simulink model "FSI_2DOF_Simscape"  (R2024a)
settings: Solver=FixedStepAuto  StartTime=0.0  StopTime=30  FixedStep=1e-4  MaxStep=1e-5  MinStep=1e-5  RelTol=1e-6  EnableMultiTasking=on
InitFcn:
  | FSI_2DOF_Simscape_init
values from neighbouring files (symbols this model uses):
  b1 = 1.5e2    (= 150)    [FSI_2DOF_Simscape_init.m]
  b2 = 5    [FSI_2DOF_Simscape_init.m]
  bias_1 = 0    [FSI_2DOF_Simscape_init.m]
  bias_2 = 0    [FSI_2DOF_Simscape_init.m]
  F_1 = 1e4    (= 10000)    [FSI_2DOF_Simscape_init.m]
  F_2 = 0    [FSI_2DOF_Simscape_init.m]
  omega_1 = 2*pi*f_1    [FSI_2DOF_Simscape_init.m]
  omega_2 = 2*pi*f_2    [FSI_2DOF_Simscape_init.m]
  phase_1 = 0    [FSI_2DOF_Simscape_init.m]
  phase_2 = 0    [FSI_2DOF_Simscape_init.m]
  t_1 = 1e-2    (= 0.01)    [FSI_2DOF_Simscape_init.m]
  t_2 = 1e-2    (= 0.01)    [FSI_2DOF_Simscape_init.m]
libraries: fl_lib x15, nesl_utility x7
settings Model: Creator=FilipKsica  LastModifiedBy=144901
settings SolverCC: InitialStep=1e-5  AlgebraicLoopSolver=TrustRegion
settings DataIOCC: LimitDataPoints=on  ReturnWorkspaceOutputs=off
settings OptimizationCC: LifeSpan=inf
settings DebuggingCC: UnconnectedInputMsg=warning  UnconnectedOutputMsg=warning  UnconnectedLineMsg=warning  AllowSymbolicDim=off  SFUnexpectedBacktrackingDiag=warning  SFNoUnconditionalDefaultTransitionDiag=warning  SFExecutionAtInitializationDiag=none  ArithmeticOperatorsInVariantConditions=warning
settings ModelReferenceCC: EnableRefExpFcnMdlSchedulingChecks=on  PropagateSignalLabelsOutOfModel=off
settings SFSimCC: SimUseLocalCustomCode=off  CustomCodeUndefinedFunction=UseInterfaceOnly
settings RTWCC: RTWUseLocalCustomCode=off  GPUComputeCapability=3.5  DLArmComputeVersion=19.05
settings CodeAppCC: StateflowObjectComments=on
settings GRTTargetCC: TargetLangStandard=C89/C90 (ANSI)
settings ConfigComp: CovMetricSettings=dw  CovSaveCumulativeToWorkspaceVar=on  CovSaveSingleToWorkspaceVar=on  CovExternalEMLEnable=off
settings SimscapeCC: SimscapeNormalizeSystem=off

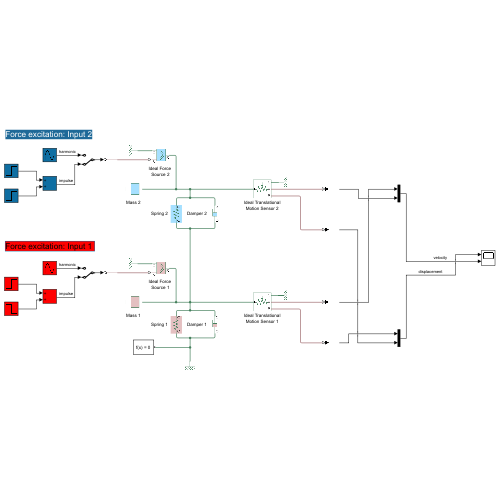
[thumbnail: Simulink's stored preview of the top-level diagram]
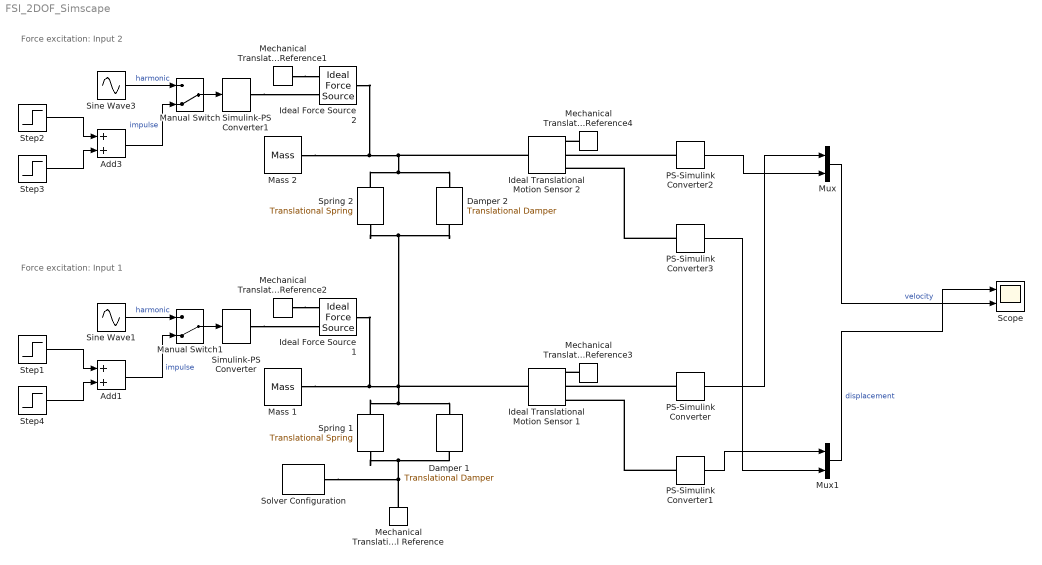
== system FSI_2DOF_Simscape ==
  note: Force excitation: Input 1
  note: Force excitation: Input 2
  Add1 : Sum
  Add3 : Sum
  Damper 1 : fl_lib/Mechanical/Translational Elements/Translational Damper  D=b1 N/(m/s)  v_specify=off  v_priority=None  v=0 m/s  v_nominal_specify=off  v_nominal_value=1  v_nominal_unit=m/s  f_specify=off  f_priority=None  f=0 N  f_nominal_specify=off  f_nominal_value=1  f_nominal_unit=N
  Damper 2 : fl_lib/Mechanical/Translational Elements/Translational Damper  D=b2 N/(m/s)  v_specify=off  v_priority=None  v=0 m/s  v_nominal_specify=off  v_nominal_value=1  v_nominal_unit=m/s  f_specify=off  f_priority=None  f=0 N  f_nominal_specify=off  f_nominal_value=1  f_nominal_unit=N
  Ideal Force Source 1 : fl_lib/Mechanical/Mechanical Sources/Ideal Force Source
  Ideal Force Source 2 : fl_lib/Mechanical/Mechanical Sources/Ideal Force Source
  Ideal Translational Motion Sensor 1 : fl_lib/Mechanical/Mechanical Sensors/Ideal Translational Motion Sensor  reference=foundation.enum.MeasurementReference.difference  acceleration_port=false  velocity_port=true  position_port=true  offset=0 m
  Ideal Translational Motion Sensor 2 : fl_lib/Mechanical/Mechanical Sensors/Ideal Translational Motion Sensor  reference=foundation.enum.MeasurementReference.difference  acceleration_port=false  velocity_port=true  position_port=true  offset=0 m
  Manual Switch : ManualSwitch  CurrentSetting=0
  Manual Switch1 : ManualSwitch  CurrentSetting=0
  Mass 1 : fl_lib/Mechanical/Translational Elements/Mass  mass=m1 kg  num_ports=foundation.enum.numPorts2.one  v_specify=off  v_priority=None  v=0 m/s  v_nominal_specify=off  v_nominal_value=1  v_nominal_unit=m/s  f_specify=off  f_priority=None  f=0 N  f_nominal_specify=off  f_nominal_value=1  f_nominal_unit=N
  Mass 2 : fl_lib/Mechanical/Translational Elements/Mass  mass=m2 kg  num_ports=foundation.enum.numPorts2.one  v_specify=off  v_priority=None  v=0 m/s  v_nominal_specify=off  v_nominal_value=1  v_nominal_unit=m/s  f_specify=off  f_priority=None  f=0 N  f_nominal_specify=off  f_nominal_value=1  f_nominal_unit=N
  Mechanical Translational Reference{,1..4} (5 alike) : fl_lib/Mechanical/Translational Elements/Mechanical Translational Reference
  Mux : Mux  Inputs=2
  Mux1 : Mux  Inputs=2
  PS-Simulink Converter{,1..3} (4 alike) : nesl_utility/PS-Simulink Converter  PhysicalDomain=network_engine_domain  SubClassName=ps_output  LeftPortType=input  RightPortType=output  PseudoPeriodic=off  Frequencies=[]  VectorFormat=1-D array  Unit=1  AffineConversion=off
  "Scope " : Scope  NumInputPorts=2
  Simulink-PS Converter : nesl_utility/Simulink-PS Converter  PhysicalDomain=network_engine_domain  SubClassName=ps_input  LeftPortType=input  RightPortType=output  PseudoPeriodic=off  Frequencies=[]  NoiseDistribution=none  NoiseParameters=[]  Unit=1  AffineConversion=off  FilteringAndDerivatives=zero  SimscapeFilterOrder=1  InputFilterTimeConstant=0.001  UdotUserProvided=1
  Simulink-PS Converter1 : nesl_utility/Simulink-PS Converter  PhysicalDomain=network_engine_domain  SubClassName=ps_input  LeftPortType=input  RightPortType=output  PseudoPeriodic=off  Frequencies=[]  NoiseDistribution=none  NoiseParameters=[]  Unit=1  AffineConversion=off  FilteringAndDerivatives=zero  SimscapeFilterOrder=1  InputFilterTimeConstant=0.001  UdotUserProvided=1
  Sine Wave1 : Sin  Amplitude=F_1  Bias=bias_1  Frequency=omega_1  Phase=phase_1  SampleTime=0
  Sine Wave3 : Sin  Amplitude=F_2  Bias=bias_2  Frequency=omega_2  Phase=phase_2  SampleTime=0
  Solver Configuration : nesl_utility/Solver Configuration  PhysicalDomain=network_engine_domain  SubClassName=solver  LeftPortType=input  RightPortType=generic  Tones=[]  Harmonics=[]  SimulateNoise=off  Profile=off  UseLocalSampling=off  EnableSwitchedLinearOptims=on  FrequencyDomain=off  UseCCode=off  RelTol=0.001  AbsTol=1e-06  MinStep=1e-09  ToWorkspace=off  RevertToSquareIcSolve=off  NumHomotopyIterations=100  PhasorMode=off  PhasorModeNumHarmonics=1  ConsistencySolver=NEWTON_FTOL  IndexReductionMethod=DerivativeReplacement  DoDC=off  ResidualTolerance=1e-09  ConsistencyTolSource=GLOBAL  ConsistencyAbsTol=0.001  ConsistencyRelTol=0.001  ConsistencyTolFactor=0.001  UseLocalSolver=off  LocalSolverChoice=NE_BACKWARD_EULER_ADVANCER  ResolveIndetEquations=on  FunctionEvalNumThread=1  LocalSolverSampleTime=0.001  DoFixedCost=off  MaxNonlinIter=3  MaxModeIter=2  ComputeImpulses=off  ImpulseIterations=2  LinearAlgebra=Sparse  LinearAlgebraNumThread=0  EquationFormulation=NE_TIME_EF  DelaysMemoryBudget=1024  AutomaticFiltering=on  FilteringTimeConstant=0.001  PartitionStorageMethod=AS_NEEDED  PartitionMemoryBudget=1024  PartitionMethod=FAST  MultibodyUseLocalSolver=off  MultibodyLocalSolverChoice=ODE1  MultibodyLocalSolverSampleTime=0.001
  Spring 1 : fl_lib/Mechanical/Translational Elements/Translational Spring  spr_rate=k1 N/m  v_specify=off  v_priority=None  v=0 m/s  v_nominal_specify=off  v_nominal_value=1  v_nominal_unit=m/s  f_specify=off  f_priority=None  f=0 N  f_nominal_specify=off  f_nominal_value=1  f_nominal_unit=N  x_specify=off  x_priority=None  x=0 m  x_nominal_specify=off  x_nominal_value=1  x_nominal_unit=m
  Spring 2 : fl_lib/Mechanical/Translational Elements/Translational Spring  spr_rate=k2 N/m  v_specify=off  v_priority=None  v=0 m/s  v_nominal_specify=off  v_nominal_value=1  v_nominal_unit=m/s  f_specify=off  f_priority=None  f=0 N  f_nominal_specify=off  f_nominal_value=1  f_nominal_unit=N  x_specify=off  x_priority=None  x=0 m  x_nominal_specify=off  x_nominal_value=1  x_nominal_unit=m
  Step1 : Step  Time=0  After=F_1  SampleTime=0
  Step2 : Step  Time=0  After=F_2  SampleTime=0
  Step3 : Step  Time=t_2  After=-F_2  SampleTime=0
  Step4 : Step  Time=t_1  After=-F_1  SampleTime=0
  wires:
  PS-Simulink Converter/1 -> Mux/1
  PS-Simulink Converter1/1 -> Mux1/1
  PS-Simulink Converter2/1 -> Mux/2
  PS-Simulink Converter3/1 -> Mux1/2
  Manual Switch1/1 -> Simulink-PS Converter/1
  Manual Switch/1 -> Simulink-PS Converter1/1
  Mux/1 -> "Scope "/2  "velocity"
  Mux1/1 -> "Scope "/1  "displacement"
  Step3/1 -> Add3/2
  Sine Wave3/1 -> Manual Switch/1  "harmonic"
  Add3/1 -> Manual Switch/2  "impulse"
  Step2/1 -> Add3/1
  Add1/1 -> Manual Switch1/2  "impulse"
  Step1/1 -> Add1/1
  Step4/1 -> Add1/2
  Sine Wave1/1 -> Manual Switch1/1  "harmonic"
  connections:
  Damper 2/RConn1 -- Spring 2/RConn1 -- Mass 1/LConn1 -- Ideal Force Source 1/LConn1 -- Ideal Translational Motion Sensor 1/LConn1 -- Spring 1/LConn1 -- Damper 1/LConn1
  Spring 1/RConn1 -- Solver Configuration/RConn1 -- Mechanical Translational Reference/LConn1 -- Damper 1/RConn1
  PS-Simulink Converter1/LConn1 -- Ideal Translational Motion Sensor 1/RConn3
  PS-Simulink Converter/LConn1 -- Ideal Translational Motion Sensor 1/RConn2
  Damper 2/LConn1 -- Ideal Translational Motion Sensor 2/LConn1 -- Mass 2/LConn1 -- Ideal Force Source 2/LConn1 -- Spring 2/LConn1
  Mechanical Translational Reference1/LConn1 -- Ideal Force Source 2/RConn2
  Mechanical Translational Reference2/LConn1 -- Ideal Force Source 1/RConn2
  Mechanical Translational Reference3/LConn1 -- Ideal Translational Motion Sensor 1/RConn1
  PS-Simulink Converter3/LConn1 -- Ideal Translational Motion Sensor 2/RConn3
  PS-Simulink Converter2/LConn1 -- Ideal Translational Motion Sensor 2/RConn2
  Mechanical Translational Reference4/LConn1 -- Ideal Translational Motion Sensor 2/RConn1
  Simulink-PS Converter/RConn1 -- Ideal Force Source 1/RConn1
  Simulink-PS Converter1/RConn1 -- Ideal Force Source 2/RConn1
